simulink model "V6_Energy_Transition_ABM"  (R2026a)
settings: Solver=FixedStepDiscrete  StartTime=0  StopTime=35  FixedStep=1
values from neighbouring files (symbols this model uses):
  V6_ANNUAL_CONTEXT = struct('parameters',input.parameters,'scenario',scenario,'mechanisms',rules,'initial_state',input.initial_state(:))    [v6_annual_run.m]
undefined symbols (not defined in the file or in its folder): v6_annual_step
Description:
  | Autonomous annual demand, generation/fuel investment, construction queues, reserves and carbon-policy feedback; fixed calibration and paid policy controls only; consumer/government/investor mechanism switches act inside native decisions, no annual replay inputs.
settings Model: Creator=Y9000P  LastModifiedBy=Y9000P

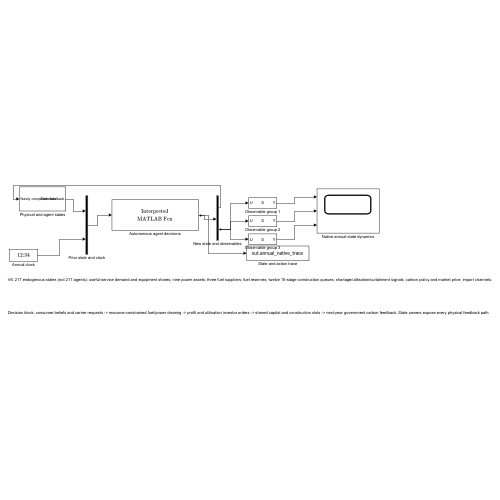
[thumbnail: Simulink's stored preview of the top-level diagram]
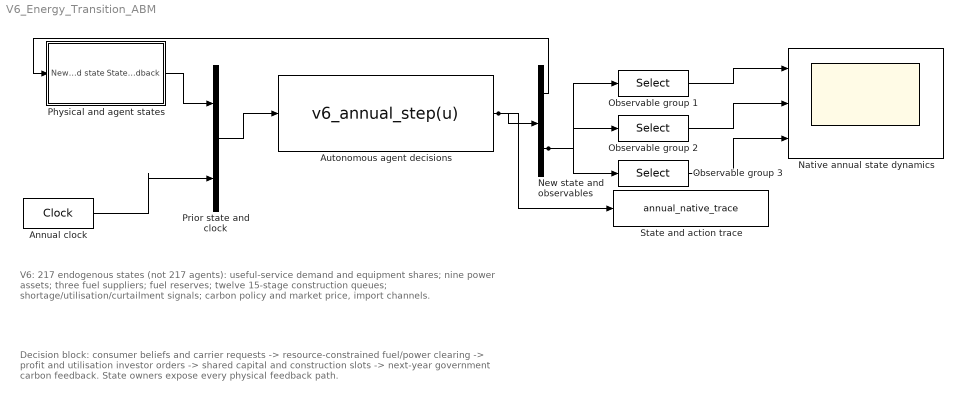
== system V6_Energy_Transition_ABM ==
  note: V6: 217 endogenous states (not 217 agents): useful-service demand and equipment shares; nine power assets; three fuel suppliers; fuel reserves; twelve 15-stage construction queues; shortage/utilisation/curtailment signals; carbon policy and market price, import channels.
  note: Decision block: consumer beliefs and carrier requests -> resource-constrained fuel/power clearing -> profit and utilisation investor orders -> shared capital and construction slots -> next-year government carbon feedback. State owners expose every physical feedback path.
  Annual clock : DigitalClock
  Autonomous agent decisions : MATLABFcn  MATLABFcn=v6_annual_step(u)  OutputDimensions=349
  Native annual state dynamics : Scope  NumInputPorts=3
  New state and observables : Demux  Outputs=[217 132]
  Observable group 1 : Selector  InputPortWidth=132  IndexOptions=Index vector (dialog)  Indices=[1 2 3]  OutputSizes=1
  Observable group 2 : Selector  InputPortWidth=132  IndexOptions=Index vector (dialog)  Indices=[5 7]  OutputSizes=1
  Observable group 3 : Selector  InputPortWidth=132  IndexOptions=Index vector (dialog)  Indices=[9 10]  OutputSizes=1
  Physical and agent states : Subsystem
  Prior state and clock : Mux  Inputs=2
  State and action trace : ToWorkspace  VariableName=annual_native_trace  SaveFormat=Structure With Time  SampleTime=-1
  wires:
  New state and observables/2 -> Observable group 1/1, Observable group 2/1, Observable group 3/1
  Observable group 1/1 -> Native annual state dynamics/1
  Observable group 2/1 -> Native annual state dynamics/2
  Observable group 3/1 -> Native annual state dynamics/3
  Physical and agent states/1(State feedback) -> Prior state and clock/1
  Annual clock/1 -> Prior state and clock/2
  Prior state and clock/1 -> Autonomous agent decisions/1
  Autonomous agent decisions/1 -> New state and observables/1, State and action trace/1
  New state and observables/1 -> Physical and agent states/1(Newly computed state)

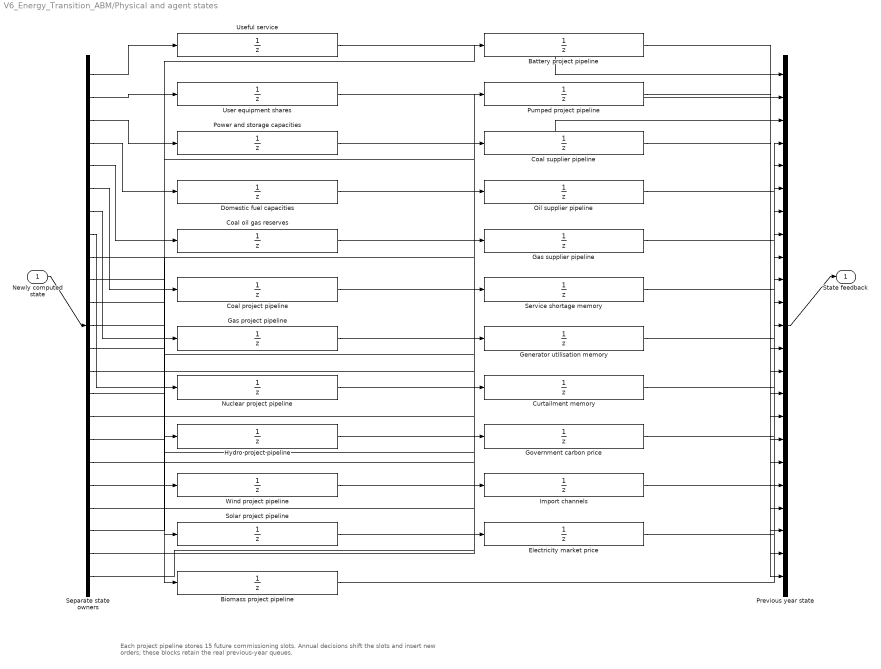
== system V6_Energy_Transition_ABM/Physical and agent states ==
  note: Each project pipeline stores 15 future commissioning slots. Annual decisions shift the slots and insert new orders; these blocks retain the real previous-year queues.
  Newly computed state : Inport
  Battery project pipeline : UnitDelay  InitialCondition=V6_ANNUAL_CONTEXT.initial_state(126:140)
  Biomass project pipeline : UnitDelay  InitialCondition=V6_ANNUAL_CONTEXT.initial_state(111:125)
  Coal oil gas reserves : UnitDelay  InitialCondition=V6_ANNUAL_CONTEXT.initial_state(18:20)
  Coal project pipeline : UnitDelay  InitialCondition=V6_ANNUAL_CONTEXT.initial_state(21:35)
  Coal supplier pipeline : UnitDelay  InitialCondition=V6_ANNUAL_CONTEXT.initial_state(156:170)
  Curtailment memory : UnitDelay  InitialCondition=V6_ANNUAL_CONTEXT.initial_state(212:212)
  Domestic fuel capacities : UnitDelay  InitialCondition=V6_ANNUAL_CONTEXT.initial_state(15:17)
  Electricity market price : UnitDelay  InitialCondition=V6_ANNUAL_CONTEXT.initial_state(217:217)
  Gas project pipeline : UnitDelay  InitialCondition=V6_ANNUAL_CONTEXT.initial_state(36:50)
  Gas supplier pipeline : UnitDelay  InitialCondition=V6_ANNUAL_CONTEXT.initial_state(186:200)
  Generator utilisation memory : UnitDelay  InitialCondition=V6_ANNUAL_CONTEXT.initial_state(205:211)
  Government carbon price : UnitDelay  InitialCondition=V6_ANNUAL_CONTEXT.initial_state(213:213)
  Hydro project pipeline : UnitDelay  InitialCondition=V6_ANNUAL_CONTEXT.initial_state(66:80)
  Import channels : UnitDelay  InitialCondition=V6_ANNUAL_CONTEXT.initial_state(214:216)
  Nuclear project pipeline : UnitDelay  InitialCondition=V6_ANNUAL_CONTEXT.initial_state(51:65)
  Oil supplier pipeline : UnitDelay  InitialCondition=V6_ANNUAL_CONTEXT.initial_state(171:185)
  Power and storage capacities : UnitDelay  InitialCondition=V6_ANNUAL_CONTEXT.initial_state(6:14)
  Previous year state : Mux  Inputs=23
  Pumped project pipeline : UnitDelay  InitialCondition=V6_ANNUAL_CONTEXT.initial_state(141:155)
  Separate state owners : Demux  Outputs=[1 4 9 3 3 15 15 15 15 15 15 15 15 15 15 15 15 4 7 1 1 3 1]
  Service shortage memory : UnitDelay  InitialCondition=V6_ANNUAL_CONTEXT.initial_state(201:204)
  Solar project pipeline : UnitDelay  InitialCondition=V6_ANNUAL_CONTEXT.initial_state(96:110)
  Useful service : UnitDelay  InitialCondition=V6_ANNUAL_CONTEXT.initial_state(1:1)
  User equipment shares : UnitDelay  InitialCondition=V6_ANNUAL_CONTEXT.initial_state(2:5)
  Wind project pipeline : UnitDelay  InitialCondition=V6_ANNUAL_CONTEXT.initial_state(81:95)
  State feedback : Outport
  wires:
  Newly computed state/1 -> Separate state owners/1
  Previous year state/1 -> State feedback/1
  Separate state owners/1 -> Useful service/1
  Useful service/1 -> Previous year state/1
  Separate state owners/2 -> User equipment shares/1
  User equipment shares/1 -> Previous year state/2
  Separate state owners/3 -> Power and storage capacities/1
  Power and storage capacities/1 -> Previous year state/3
  Separate state owners/4 -> Domestic fuel capacities/1
  Domestic fuel capacities/1 -> Previous year state/4
  Separate state owners/5 -> Coal oil gas reserves/1
  Coal oil gas reserves/1 -> Previous year state/5
  Separate state owners/6 -> Coal project pipeline/1
  Coal project pipeline/1 -> Previous year state/6
  Separate state owners/7 -> Gas project pipeline/1
  Gas project pipeline/1 -> Previous year state/7
  Separate state owners/8 -> Nuclear project pipeline/1
  Nuclear project pipeline/1 -> Previous year state/8
  Separate state owners/9 -> Hydro project pipeline/1
  Hydro project pipeline/1 -> Previous year state/9
  Separate state owners/10 -> Wind project pipeline/1
  Wind project pipeline/1 -> Previous year state/10
  Separate state owners/11 -> Solar project pipeline/1
  Solar project pipeline/1 -> Previous year state/11
  Separate state owners/12 -> Biomass project pipeline/1
  Biomass project pipeline/1 -> Previous year state/12
  Separate state owners/13 -> Battery project pipeline/1
  Battery project pipeline/1 -> Previous year state/13
  Separate state owners/14 -> Pumped project pipeline/1
  Pumped project pipeline/1 -> Previous year state/14
  Separate state owners/15 -> Coal supplier pipeline/1
  Coal supplier pipeline/1 -> Previous year state/15
  Separate state owners/16 -> Oil supplier pipeline/1
  Oil supplier pipeline/1 -> Previous year state/16
  Separate state owners/17 -> Gas supplier pipeline/1
  Gas supplier pipeline/1 -> Previous year state/17
  Separate state owners/18 -> Service shortage memory/1
  Service shortage memory/1 -> Previous year state/18
  Separate state owners/19 -> Generator utilisation memory/1
  Generator utilisation memory/1 -> Previous year state/19
  Separate state owners/20 -> Curtailment memory/1
  Curtailment memory/1 -> Previous year state/20
  Separate state owners/21 -> Government carbon price/1
  Government carbon price/1 -> Previous year state/21
  Separate state owners/22 -> Import channels/1
  Import channels/1 -> Previous year state/22
  Separate state owners/23 -> Electricity market price/1
  Electricity market price/1 -> Previous year state/23
